simulink model "DroneFlight"  (Simulink 8.0)
settings: Solver=ode4  SolverType=Fixed-step  StopTime=9  FixedStep=drone.step_s
InitFcn:
  | setup_flight;
undefined symbols (not defined in the file): drone
settings Model: ReturnWorkspaceOutputs=on

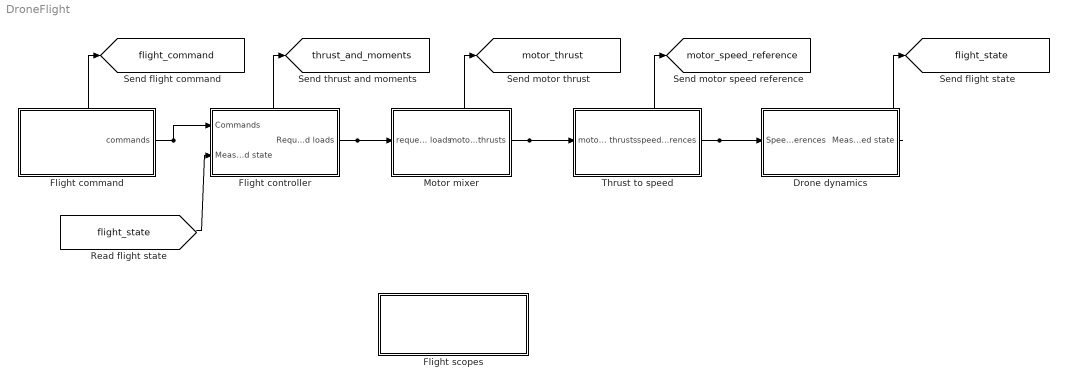
== system DroneFlight ==
  Flight command : Subsystem
  Flight controller : Subsystem
  Motor mixer : Subsystem
  Thrust to speed : Subsystem
  Drone dynamics : Subsystem
  Flight scopes : Subsystem
  tag scope: flight_command=global, flight_state=global, motor_speed_reference=global, motor_thrust=global, thrust_and_moments=global
  wires:
  Flight command/1(commands) -> Flight controller/1(Commands), [flight_command]
  Flight controller/1(Requested loads) -> Motor mixer/1(requested loads), [thrust_and_moments]
  Motor mixer/1(motor thrusts) -> Thrust to speed/1(motor thrusts), [motor_thrust]
  Thrust to speed/1(speed references) -> Drone dynamics/1(Speed references), [motor_speed_reference]
  Drone dynamics/1(Measured state) -> [flight_state]
  [flight_state] -> Flight controller/2(Measured state)

== system DroneFlight/Flight command ==
  Forward speed command : FromWorkspace  VariableName=forward_command  Interpolate=off  OutputAfterFinalValue=Holding final value  SampleTime=drone.step_s
  Right climb height and yaw : FromWorkspace  VariableName=mission_commands  Interpolate=off  OutputAfterFinalValue=Holding final value  SampleTime=drone.step_s
  Collect commands : Mux  Inputs=2
  commands : Outport  Port=1
  wires:
  Forward speed command/1 -> Collect commands/1  "Forward speed (m per s)"
  Right climb height and yaw/1 -> Collect commands/2
  Collect commands/1 -> commands/1

== system DroneFlight/Flight controller ==
  Commands : Inport  Port=1
  Measured state : Inport  Port=2
  Movement references : Demux  Outputs=[2 1 1 1]
  Feedback channels : Demux  Outputs=[2 1 2 1 2 1 3 4]
  Feedback channels unused 1 : Terminator
  Feedback channels unused 8 : Terminator
  Horizontal velocity : Subsystem
  Height and climb : Subsystem
  Attitude and body rates : Subsystem
  Collective roll pitch yaw : Mux  Inputs=2
  Requested loads : Outport  Port=1
  wires:
  Commands/1 -> Movement references/1
  Measured state/1 -> Feedback channels/1
  Feedback channels/1 -> Feedback channels unused 1/1
  Feedback channels/8 -> Feedback channels unused 8/1
  Movement references/1 -> Horizontal velocity/1(Forward and right demand)
  Feedback channels/3 -> Horizontal velocity/2(North and east velocity)
  Feedback channels/6 -> Horizontal velocity/3(Heading)
  Movement references/2 -> Height and climb/1(Climb demand)
  Movement references/3 -> Height and climb/2(Height demand)
  Feedback channels/2 -> Height and climb/3(Down position)
  Feedback channels/4 -> Height and climb/4(Down velocity)
  Feedback channels/5 -> Height and climb/5(Roll and pitch), Attitude and body rates/2(Measured roll and pitch)
  Horizontal velocity/1(Roll and pitch demand) -> Attitude and body rates/1(Demanded roll and pitch)
  Movement references/4 -> Attitude and body rates/3(Demanded yaw rate)
  Feedback channels/7 -> Attitude and body rates/4(Body rates)
  Height and climb/1(Collective thrust) -> Collective roll pitch yaw/1
  Attitude and body rates/1(Body moments) -> Collective roll pitch yaw/2
  Collective roll pitch yaw/1 -> Requested loads/1

== system DroneFlight/Motor mixer ==
  requested loads : Inport  Port=1
  Mix thrust and moments : Gain  Gain=drone.allocation  Multiplication=Matrix(K*u)
  Rotor thrust limits : Subsystem
  motor thrusts : Outport  Port=1
  wires:
  requested loads/1 -> Mix thrust and moments/1
  Mix thrust and moments/1 -> Rotor thrust limits/1(Raw rotor thrusts)
  Rotor thrust limits/1(Feasible thrusts) -> motor thrusts/1

== system DroneFlight/Thrust to speed ==
  motor thrusts : Inport  Port=1
  Inverse thrust coefficient : Gain  Gain=1/drone.kT
  Square root : Sqrt
  speed references : Outport  Port=1
  wires:
  motor thrusts/1 -> Inverse thrust coefficient/1
  Inverse thrust coefficient/1 -> Square root/1
  Square root/1 -> speed references/1

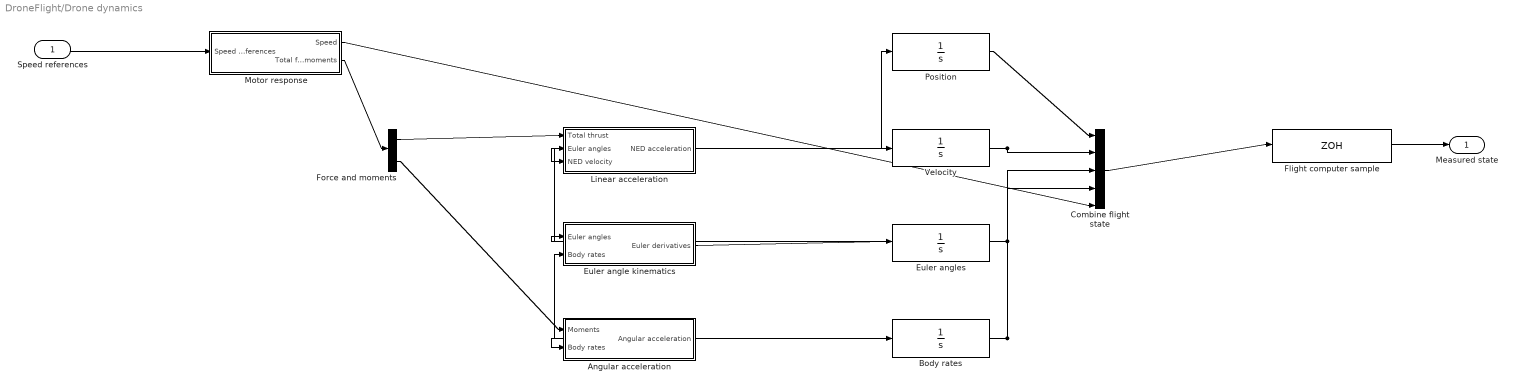
== system DroneFlight/Drone dynamics ==
  Speed references : Inport  Port=1
  Motor response : Subsystem
  Force and moments : Demux  Outputs=[1 3]
  Position : Integrator  InitialCondition=drone.x0(1:3)
  Velocity : Integrator  InitialCondition=drone.x0(4:6)
  Euler angles : Integrator  InitialCondition=drone.x0(7:9)
  Body rates : Integrator  InitialCondition=drone.x0(10:12)
  Linear acceleration : Subsystem
  Euler angle kinematics : Subsystem
  Angular acceleration : Subsystem
  Combine flight state : Mux  Inputs=5
  Flight computer sample : ZeroOrderHold  SampleTime=drone.step_s
  Measured state : Outport  Port=1
  wires:
  Speed references/1 -> Motor response/1(Speed references)
  Motor response/2(Total force and moments) -> Force and moments/1
  Force and moments/1 -> Linear acceleration/1(Total thrust)
  Euler angles/1 -> Linear acceleration/2(Euler angles), Euler angle kinematics/1(Euler angles), Combine flight state/3
  Velocity/1 -> Linear acceleration/3(NED velocity), Position/1, Combine flight state/2
  Body rates/1 -> Euler angle kinematics/2(Body rates), Angular acceleration/2(Body rates), Combine flight state/4
  Force and moments/2 -> Angular acceleration/1(Moments)
  Linear acceleration/1(NED acceleration) -> Velocity/1
  Euler angle kinematics/1(Euler derivatives) -> Euler angles/1
  Angular acceleration/1(Angular acceleration) -> Body rates/1
  Position/1 -> Combine flight state/1
  Motor response/1(Speed) -> Combine flight state/5
  Combine flight state/1 -> Flight computer sample/1
  Flight computer sample/1 -> Measured state/1

== system DroneFlight/Flight scopes ==
  Flight response : Subsystem
  Mixer inputs : Subsystem
  Motor outputs : Subsystem
  Flight measurements : Subsystem
  wires:
  [flight_command] -> Flight response/1(Reference)
  [flight_state] -> Flight measurements/1(State)
  [thrust_and_moments] -> Mixer inputs/1(Controller request)
  [motor_thrust] -> Motor outputs/1(Thrust references)
  [motor_speed_reference] -> Motor outputs/2(Speed references)
  Flight measurements/1(Measurements) -> Flight response/2(Instruments), Motor outputs/3(Instruments)

== system DroneFlight/Flight controller/Horizontal velocity ==
  Forward and right demand : Inport  Port=1
  North and east velocity : Inport  Port=2
  Heading : Inport  Port=3
  Rotate velocity into body : Subsystem
  Velocity error : Sum  Inputs=+-
  Velocity gain : Gain  Gain=drone.velocity_gain_per_s
  Drag feedforward : Gain  Gain=drone.linear_drag_N_per_m_s/drone.mass_kg
  Requested acceleration : Sum  Inputs=++
  Bound horizontal acceleration : Subsystem
  Convert acceleration to tilt : Subsystem
  Roll and pitch demand : Outport  Port=1
  wires:
  North and east velocity/1 -> Rotate velocity into body/1(Planar components)
  Heading/1 -> Rotate velocity into body/2(Yaw)
  Forward and right demand/1 -> Velocity error/1, Drag feedforward/1
  Rotate velocity into body/1(Rotated vector) -> Velocity error/2
  Velocity error/1 -> Velocity gain/1
  Velocity gain/1 -> Requested acceleration/1
  Drag feedforward/1 -> Requested acceleration/2
  Requested acceleration/1 -> Bound horizontal acceleration/1(Acceleration)
  Bound horizontal acceleration/1(Bounded acceleration) -> Convert acceleration to tilt/1(Forward and right acceleration)
  Convert acceleration to tilt/1(Roll and pitch) -> Roll and pitch demand/1

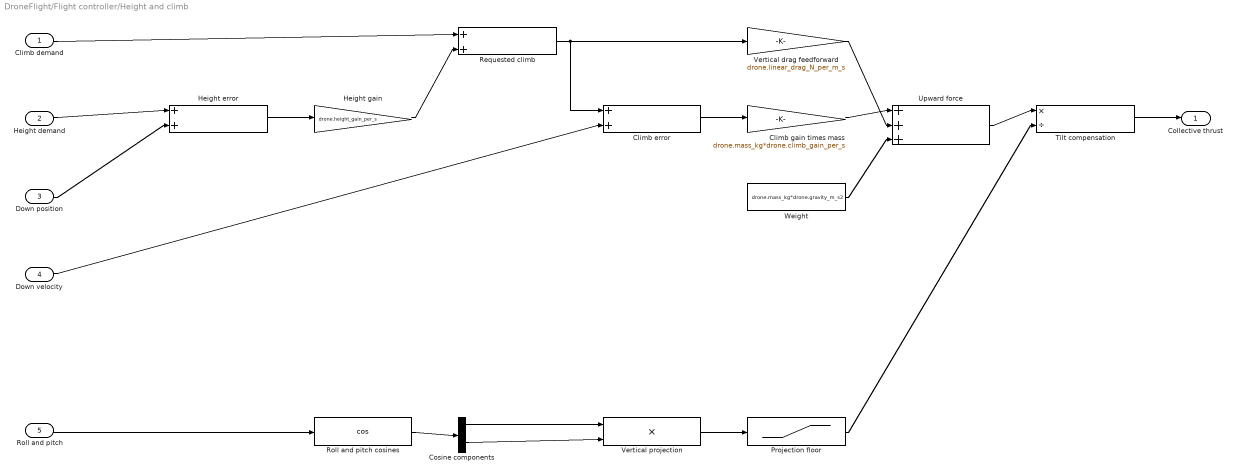
== system DroneFlight/Flight controller/Height and climb ==
  Climb demand : Inport  Port=1
  Height demand : Inport  Port=2
  Down position : Inport  Port=3
  Down velocity : Inport  Port=4
  Roll and pitch : Inport  Port=5
  Height error : Sum  Inputs=++
  Height gain : Gain  Gain=drone.height_gain_per_s
  Requested climb : Sum  Inputs=++
  Climb error : Sum  Inputs=++
  Climb gain times mass : Gain  Gain=drone.mass_kg*drone.climb_gain_per_s
  Vertical drag feedforward : Gain  Gain=drone.linear_drag_N_per_m_s
  Weight : Constant  Value=drone.mass_kg*drone.gravity_m_s2
  Upward force : Sum  Inputs=+++
  Roll and pitch cosines : Trigonometry  Operator=cos
  Cosine components : Demux  Outputs=[1 1]
  Vertical projection : Product  Inputs=**
  Projection floor : Saturate  LowerLimit=0.5  UpperLimit=1
  Tilt compensation : Product  Inputs=*/
  Collective thrust : Outport  Port=1
  wires:
  Height demand/1 -> Height error/1
  Down position/1 -> Height error/2
  Height error/1 -> Height gain/1
  Climb demand/1 -> Requested climb/1
  Height gain/1 -> Requested climb/2
  Requested climb/1 -> Climb error/1, Vertical drag feedforward/1
  Down velocity/1 -> Climb error/2
  Climb error/1 -> Climb gain times mass/1
  Climb gain times mass/1 -> Upward force/1
  Vertical drag feedforward/1 -> Upward force/2
  Weight/1 -> Upward force/3
  Roll and pitch/1 -> Roll and pitch cosines/1
  Roll and pitch cosines/1 -> Cosine components/1
  Cosine components/1 -> Vertical projection/1
  Cosine components/2 -> Vertical projection/2
  Vertical projection/1 -> Projection floor/1
  Upward force/1 -> Tilt compensation/1
  Projection floor/1 -> Tilt compensation/2
  Tilt compensation/1 -> Collective thrust/1

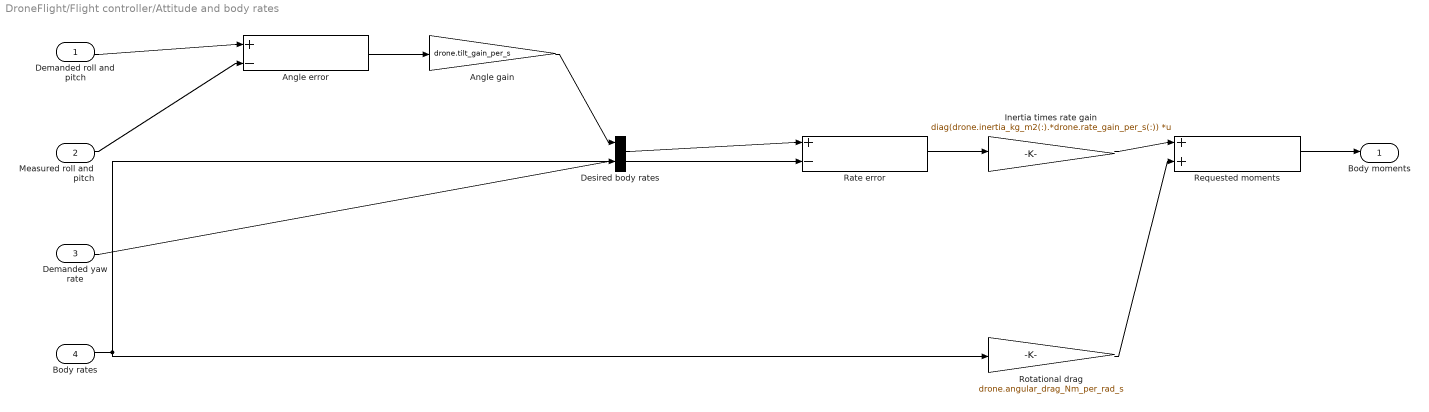
== system DroneFlight/Flight controller/Attitude and body rates ==
  Demanded roll and pitch : Inport  Port=1
  Measured roll and pitch : Inport  Port=2
  Demanded yaw rate : Inport  Port=3
  Body rates : Inport  Port=4
  Angle error : Sum  Inputs=+-
  Angle gain : Gain  Gain=drone.tilt_gain_per_s
  Desired body rates : Mux  Inputs=2
  Rate error : Sum  Inputs=+-
  Inertia times rate gain : Gain  Gain=diag(drone.inertia_kg_m2(:).*drone.rate_gain_per_s(:))  Multiplication=Matrix(K*u)
  Rotational drag : Gain  Gain=drone.angular_drag_Nm_per_rad_s
  Requested moments : Sum  Inputs=++
  Body moments : Outport  Port=1
  wires:
  Demanded roll and pitch/1 -> Angle error/1
  Measured roll and pitch/1 -> Angle error/2
  Angle error/1 -> Angle gain/1
  Angle gain/1 -> Desired body rates/1
  Demanded yaw rate/1 -> Desired body rates/2
  Desired body rates/1 -> Rate error/1
  Body rates/1 -> Rate error/2, Rotational drag/1
  Rate error/1 -> Inertia times rate gain/1
  Inertia times rate gain/1 -> Requested moments/1
  Rotational drag/1 -> Requested moments/2
  Requested moments/1 -> Body moments/1

== system DroneFlight/Motor mixer/Rotor thrust limits ==
  Raw rotor thrusts : Inport  Port=1
  Mean rotor thrust : Gain  Gain=ones(1,4)/4  Multiplication=Matrix(K*u)
  Available collective : Saturate  LowerLimit=0  UpperLimit=drone.max_thrust
  Differential thrusts : Sum  Inputs=+-
  Scale to motor limits : Subsystem
  Scale differences : Product  Inputs=**
  Restore collective : Sum  Inputs=++
  Thrust bounds : Saturate  LowerLimit=0  UpperLimit=drone.max_thrust
  Feasible thrusts : Outport  Port=1
  wires:
  Raw rotor thrusts/1 -> Mean rotor thrust/1, Differential thrusts/1
  Mean rotor thrust/1 -> Available collective/1, Differential thrusts/2
  Differential thrusts/1 -> Scale to motor limits/1(Differential thrusts), Scale differences/1
  Available collective/1 -> Scale to motor limits/2(Collective per rotor), Restore collective/1
  Scale to motor limits/1(Scale) -> Scale differences/2
  Scale differences/1 -> Restore collective/2
  Restore collective/1 -> Thrust bounds/1
  Thrust bounds/1 -> Feasible thrusts/1

== system DroneFlight/Drone dynamics/Motor response ==
  Speed references : Inport  Port=1
  Rotor speed : Integrator  InitialCondition=drone.x0(13:16)
  Speed error : Sum  Inputs=+-
  Inverse motor time constant : Gain  Gain=1/drone.speed_lag_s
  Speed : Outport  Port=1
  Speed squared : Product  Inputs=**
  Propeller thrust : Gain  Gain=drone.kT
  Thrust to body loads : Gain  Gain=drone.effectiveness  Multiplication=Matrix(K*u)
  Total force and moments : Outport  Port=2
  wires:
  Speed references/1 -> Speed error/1
  Rotor speed/1 -> Speed error/2, Speed/1, Speed squared/1, Speed squared/2
  Speed error/1 -> Inverse motor time constant/1
  Inverse motor time constant/1 -> Rotor speed/1
  Speed squared/1 -> Propeller thrust/1
  Propeller thrust/1 -> Thrust to body loads/1
  Thrust to body loads/1 -> Total force and moments/1

== system DroneFlight/Drone dynamics/Linear acceleration ==
  Total thrust : Inport  Port=1
  Euler angles : Inport  Port=2
  NED velocity : Inport  Port=3
  Body thrust direction : Subsystem
  Thrust along body down : Product  Inputs=**
  Linear drag : Gain  Gain=drone.linear_drag_N_per_m_s
  Thrust and drag : Sum  Inputs=++
  Force to acceleration : Gain  Gain=1/drone.mass_kg
  NED gravity : Constant  Value=[0;0;drone.gravity_m_s2]
  Gravity minus thrust and drag : Sum  Inputs=+-
  NED acceleration : Outport  Port=1
  wires:
  Euler angles/1 -> Body thrust direction/1(Euler angles)
  Total thrust/1 -> Thrust along body down/1
  Body thrust direction/1(Body down axis in NED) -> Thrust along body down/2
  NED velocity/1 -> Linear drag/1
  Thrust along body down/1 -> Thrust and drag/1
  Linear drag/1 -> Thrust and drag/2
  Thrust and drag/1 -> Force to acceleration/1
  NED gravity/1 -> Gravity minus thrust and drag/1
  Force to acceleration/1 -> Gravity minus thrust and drag/2
  Gravity minus thrust and drag/1 -> NED acceleration/1

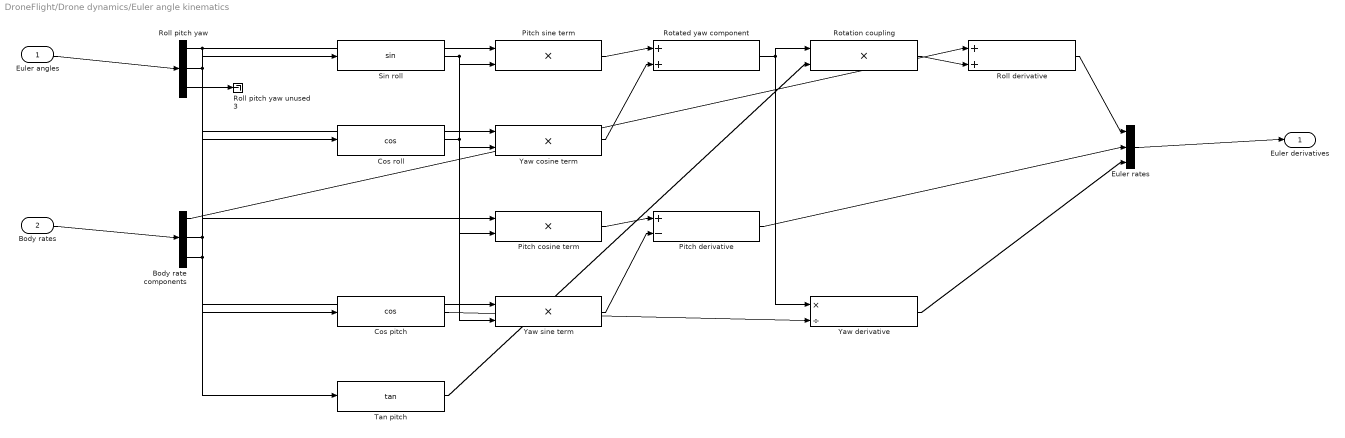
== system DroneFlight/Drone dynamics/Euler angle kinematics ==
  Euler angles : Inport  Port=1
  Body rates : Inport  Port=2
  Roll pitch yaw : Demux  Outputs=[1 1 1]
  Roll pitch yaw unused 3 : Terminator
  Body rate components : Demux  Outputs=[1 1 1]
  Sin roll : Trigonometry  Operator=sin
  Cos roll : Trigonometry  Operator=cos
  Cos pitch : Trigonometry  Operator=cos
  Tan pitch : Trigonometry  Operator=tan
  Pitch sine term : Product  Inputs=**
  Yaw cosine term : Product  Inputs=**
  Pitch cosine term : Product  Inputs=**
  Yaw sine term : Product  Inputs=**
  Rotated yaw component : Sum  Inputs=++
  Pitch derivative : Sum  Inputs=+-
  Rotation coupling : Product  Inputs=**
  Yaw derivative : Product  Inputs=*/
  Roll derivative : Sum  Inputs=++
  Euler rates : Mux  Inputs=3
  Euler derivatives : Outport  Port=1
  wires:
  Euler angles/1 -> Roll pitch yaw/1
  Roll pitch yaw/3 -> Roll pitch yaw unused 3/1
  Body rates/1 -> Body rate components/1
  Roll pitch yaw/1 -> Sin roll/1, Cos roll/1
  Roll pitch yaw/2 -> Cos pitch/1, Tan pitch/1
  Body rate components/2 -> Pitch sine term/1, Pitch cosine term/1
  Sin roll/1 -> Pitch sine term/2, Yaw sine term/2
  Body rate components/3 -> Yaw cosine term/1, Yaw sine term/1
  Cos roll/1 -> Yaw cosine term/2, Pitch cosine term/2
  Pitch sine term/1 -> Rotated yaw component/1
  Yaw cosine term/1 -> Rotated yaw component/2
  Pitch cosine term/1 -> Pitch derivative/1
  Yaw sine term/1 -> Pitch derivative/2
  Rotated yaw component/1 -> Rotation coupling/1, Yaw derivative/1
  Tan pitch/1 -> Rotation coupling/2
  Cos pitch/1 -> Yaw derivative/2
  Body rate components/1 -> Roll derivative/1
  Rotation coupling/1 -> Roll derivative/2
  Roll derivative/1 -> Euler rates/1
  Pitch derivative/1 -> Euler rates/2
  Yaw derivative/1 -> Euler rates/3
  Euler rates/1 -> Euler derivatives/1

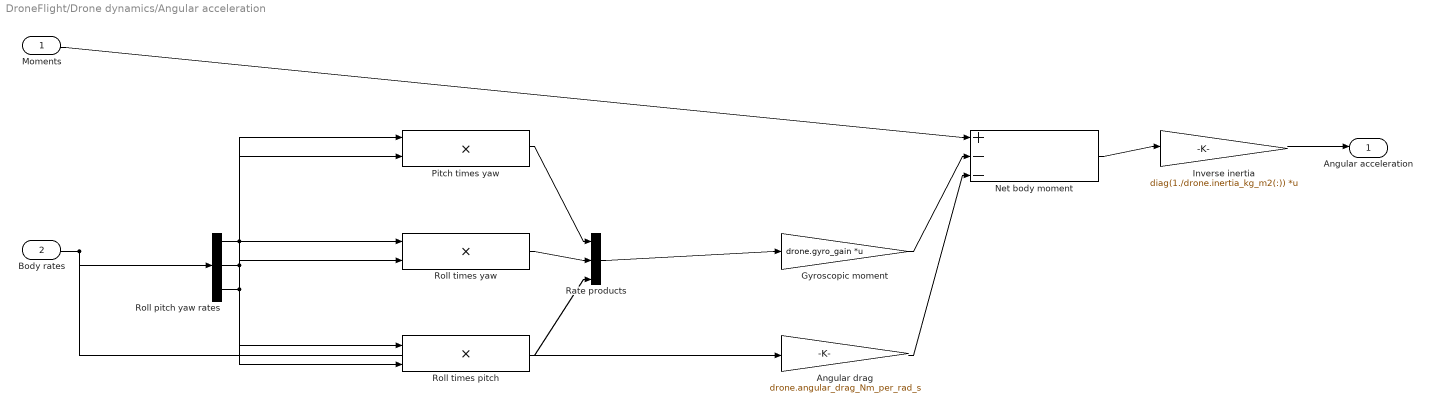
== system DroneFlight/Drone dynamics/Angular acceleration ==
  Moments : Inport  Port=1
  Body rates : Inport  Port=2
  Roll pitch yaw rates : Demux  Outputs=[1 1 1]
  Pitch times yaw : Product  Inputs=**
  Roll times yaw : Product  Inputs=**
  Roll times pitch : Product  Inputs=**
  Rate products : Mux  Inputs=3
  Gyroscopic moment : Gain  Gain=drone.gyro_gain  Multiplication=Matrix(K*u)
  Angular drag : Gain  Gain=drone.angular_drag_Nm_per_rad_s
  Net body moment : Sum  Inputs=+--
  Inverse inertia : Gain  Gain=diag(1./drone.inertia_kg_m2(:))  Multiplication=Matrix(K*u)
  Angular acceleration : Outport  Port=1
  wires:
  Body rates/1 -> Roll pitch yaw rates/1, Angular drag/1
  Roll pitch yaw rates/2 -> Pitch times yaw/1, Roll times pitch/2
  Roll pitch yaw rates/3 -> Pitch times yaw/2, Roll times yaw/2
  Roll pitch yaw rates/1 -> Roll times yaw/1, Roll times pitch/1
  Pitch times yaw/1 -> Rate products/1
  Roll times yaw/1 -> Rate products/2
  Roll times pitch/1 -> Rate products/3
  Rate products/1 -> Gyroscopic moment/1
  Moments/1 -> Net body moment/1
  Gyroscopic moment/1 -> Net body moment/2
  Angular drag/1 -> Net body moment/3
  Net body moment/1 -> Inverse inertia/1
  Inverse inertia/1 -> Angular acceleration/1

== system DroneFlight/Flight scopes/Flight response ==
  Reference : Inport  Port=1
  Instruments : Inport  Port=2
  Reference channels : Demux  Outputs=[1 2 1 1]
  Reference channels unused 2 : Terminator
  Reference channels unused 4 : Terminator
  Measured channels : Demux  Outputs=[1 1 2 3 8]
  Measured channels unused 5 : Terminator
  Forward speed - m per s : Scope  NumInputPorts=2
      settings: OpenAtSimulationStart=off
  Height - m : Scope  NumInputPorts=2
      settings: OpenAtSimulationStart=off
  North and east - m : Scope
      settings: OpenAtSimulationStart=off
  Roll pitch yaw - deg : Scope
      settings: OpenAtSimulationStart=off
  wires:
  Reference/1 -> Reference channels/1
  Reference channels/2 -> Reference channels unused 2/1
  Reference channels/4 -> Reference channels unused 4/1
  Instruments/1 -> Measured channels/1
  Measured channels/5 -> Measured channels unused 5/1
  Reference channels/1 -> Forward speed - m per s/1  "Command"
  Measured channels/1 -> Forward speed - m per s/2  "Actual"
  Reference channels/3 -> Height - m/1  "Target height"
  Measured channels/2 -> Height - m/2  "Measured height"
  Measured channels/3 -> North and east - m/1
  Measured channels/4 -> Roll pitch yaw - deg/1

== system DroneFlight/Flight scopes/Mixer inputs ==
  Controller request : Inport  Port=1
  Force and moments : Demux  Outputs=[1 3]
  Collective thrust - N : Scope
      settings: OpenAtSimulationStart=off
  Roll pitch yaw moments - Nm : Scope
      settings: OpenAtSimulationStart=off
  wires:
  Controller request/1 -> Force and moments/1
  Force and moments/1 -> Collective thrust - N/1
  Force and moments/2 -> Roll pitch yaw moments - Nm/1

== system DroneFlight/Flight scopes/Motor outputs ==
  Thrust references : Inport  Port=1
  Speed references : Inport  Port=2
  Instruments : Inport  Port=3
  Four thrust references - N channels : Demux  Outputs=[1 1 1 1]
  Four thrust references - N : Scope  NumInputPorts=4
      settings: OpenAtSimulationStart=off
  Radians per second to rpm : Gain  Gain=30/pi
  Four speed references - rpm channels : Demux  Outputs=[1 1 1 1]
  Four speed references - rpm : Scope  NumInputPorts=4
      settings: OpenAtSimulationStart=off
  Motor measurements : Demux  Outputs=[7 4 4]
  Motor measurements unused 1 : Terminator
  Actual rotor speeds - rpm : Scope
      settings: OpenAtSimulationStart=off
  Propeller loads - Nm : Scope
      settings: OpenAtSimulationStart=off
  wires:
  Thrust references/1 -> Four thrust references - N channels/1
  Four thrust references - N channels/1 -> Four thrust references - N/1  "M1 front right N"
  Four thrust references - N channels/2 -> Four thrust references - N/2  "M2 back left N"
  Four thrust references - N channels/3 -> Four thrust references - N/3  "M3 front left N"
  Four thrust references - N channels/4 -> Four thrust references - N/4  "M4 back right N"
  Speed references/1 -> Radians per second to rpm/1
  Radians per second to rpm/1 -> Four speed references - rpm channels/1
  Four speed references - rpm channels/1 -> Four speed references - rpm/1  "M1 front right rpm"
  Four speed references - rpm channels/2 -> Four speed references - rpm/2  "M2 back left rpm"
  Four speed references - rpm channels/3 -> Four speed references - rpm/3  "M3 front left rpm"
  Four speed references - rpm channels/4 -> Four speed references - rpm/4  "M4 back right rpm"
  Instruments/1 -> Motor measurements/1
  Motor measurements/1 -> Motor measurements unused 1/1
  Motor measurements/2 -> Actual rotor speeds - rpm/1
  Motor measurements/3 -> Propeller loads - Nm/1

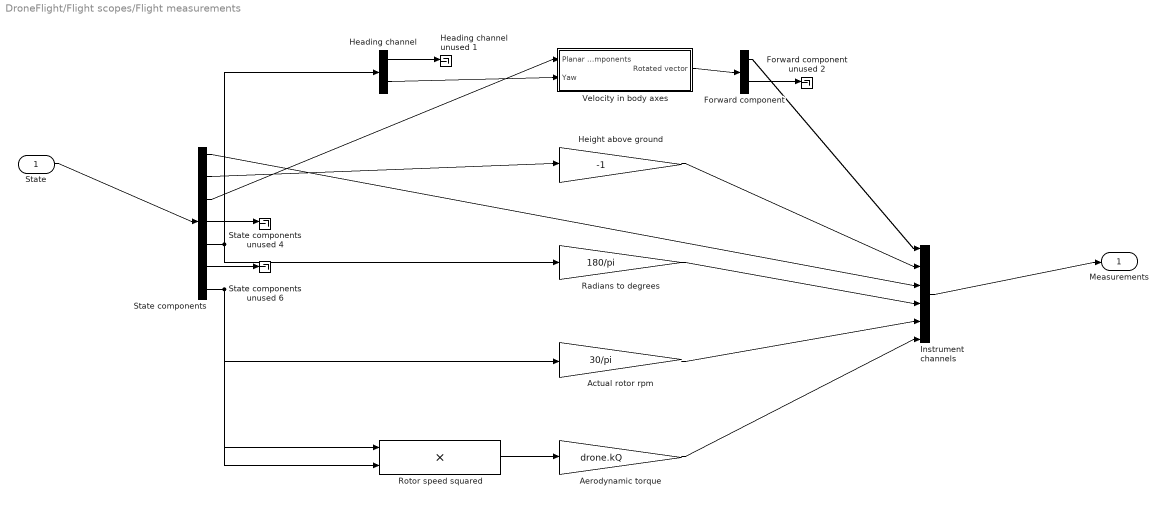
== system DroneFlight/Flight scopes/Flight measurements ==
  State : Inport  Port=1
  State components : Demux  Outputs=[2 1 2 1 3 3 4]
  State components unused 4 : Terminator
  State components unused 6 : Terminator
  Heading channel : Demux  Outputs=[2 1]
  Heading channel unused 1 : Terminator
  Velocity in body axes : Subsystem
  Forward component : Demux  Outputs=[1 1]
  Forward component unused 2 : Terminator
  Height above ground : Gain  Gain=-1
  Radians to degrees : Gain  Gain=180/pi
  Actual rotor rpm : Gain  Gain=30/pi
  Rotor speed squared : Product  Inputs=**
  Aerodynamic torque : Gain  Gain=drone.kQ
  Instrument channels : Mux  Inputs=6
  Measurements : Outport  Port=1
  wires:
  State/1 -> State components/1
  State components/4 -> State components unused 4/1
  State components/6 -> State components unused 6/1
  State components/5 -> Heading channel/1, Radians to degrees/1
  Heading channel/1 -> Heading channel unused 1/1
  State components/3 -> Velocity in body axes/1(Planar components)
  Heading channel/2 -> Velocity in body axes/2(Yaw)
  Velocity in body axes/1(Rotated vector) -> Forward component/1
  Forward component/2 -> Forward component unused 2/1
  State components/2 -> Height above ground/1
  State components/7 -> Actual rotor rpm/1, Rotor speed squared/1, Rotor speed squared/2
  Rotor speed squared/1 -> Aerodynamic torque/1
  Forward component/1 -> Instrument channels/1
  Height above ground/1 -> Instrument channels/2
  State components/1 -> Instrument channels/3
  Radians to degrees/1 -> Instrument channels/4
  Actual rotor rpm/1 -> Instrument channels/5
  Aerodynamic torque/1 -> Instrument channels/6
  Instrument channels/1 -> Measurements/1

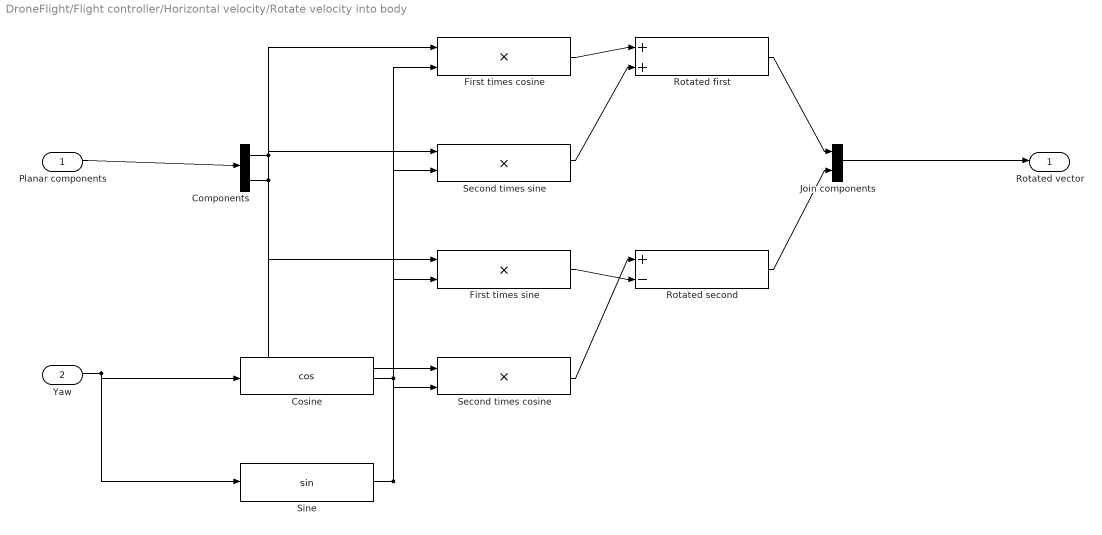
== system DroneFlight/Flight controller/Horizontal velocity/Rotate velocity into body ==
  Planar components : Inport  Port=1
  Components : Demux  Outputs=[1 1]
  Yaw : Inport  Port=2
  Cosine : Trigonometry  Operator=cos
  Sine : Trigonometry  Operator=sin
  First times cosine : Product  Inputs=**
  Second times sine : Product  Inputs=**
  First times sine : Product  Inputs=**
  Second times cosine : Product  Inputs=**
  Rotated first : Sum  Inputs=++
  Rotated second : Sum  Inputs=+-
  Join components : Mux  Inputs=2
  Rotated vector : Outport  Port=1
  wires:
  Planar components/1 -> Components/1
  Yaw/1 -> Cosine/1, Sine/1
  Components/1 -> First times cosine/1, First times sine/1
  Cosine/1 -> First times cosine/2, Second times cosine/2
  Components/2 -> Second times sine/1, Second times cosine/1
  Sine/1 -> Second times sine/2, First times sine/2
  First times cosine/1 -> Rotated first/1
  Second times sine/1 -> Rotated first/2
  Second times cosine/1 -> Rotated second/1
  First times sine/1 -> Rotated second/2
  Rotated first/1 -> Join components/1
  Rotated second/1 -> Join components/2
  Join components/1 -> Rotated vector/1

== system DroneFlight/Flight controller/Horizontal velocity/Bound horizontal acceleration ==
  Acceleration : Inport  Port=1
  Squared magnitude : DotProduct
  Magnitude : Sqrt
  Relative to limit : Gain  Gain=1/drone.max_accel_m_s2
  Minimum divisor of one : Saturate  LowerLimit=1  UpperLimit=inf
  Scale vector : Product  Inputs=*/
  Bounded acceleration : Outport  Port=1
  wires:
  Acceleration/1 -> Squared magnitude/1, Squared magnitude/2, Scale vector/1
  Squared magnitude/1 -> Magnitude/1
  Magnitude/1 -> Relative to limit/1
  Relative to limit/1 -> Minimum divisor of one/1
  Minimum divisor of one/1 -> Scale vector/2
  Scale vector/1 -> Bounded acceleration/1

== system DroneFlight/Flight controller/Horizontal velocity/Convert acceleration to tilt ==
  Forward and right acceleration : Inport  Port=1
  Divide by gravity : Gain  Gain=1/drone.gravity_m_s2
  Tilt angles : Trigonometry  Operator=atan
  Right to roll and forward to pitch : Gain  Gain=[0 1;-1 0]  Multiplication=Matrix(K*u)
  Roll and pitch : Outport  Port=1
  wires:
  Forward and right acceleration/1 -> Divide by gravity/1
  Divide by gravity/1 -> Tilt angles/1
  Tilt angles/1 -> Right to roll and forward to pitch/1
  Right to roll and forward to pitch/1 -> Roll and pitch/1

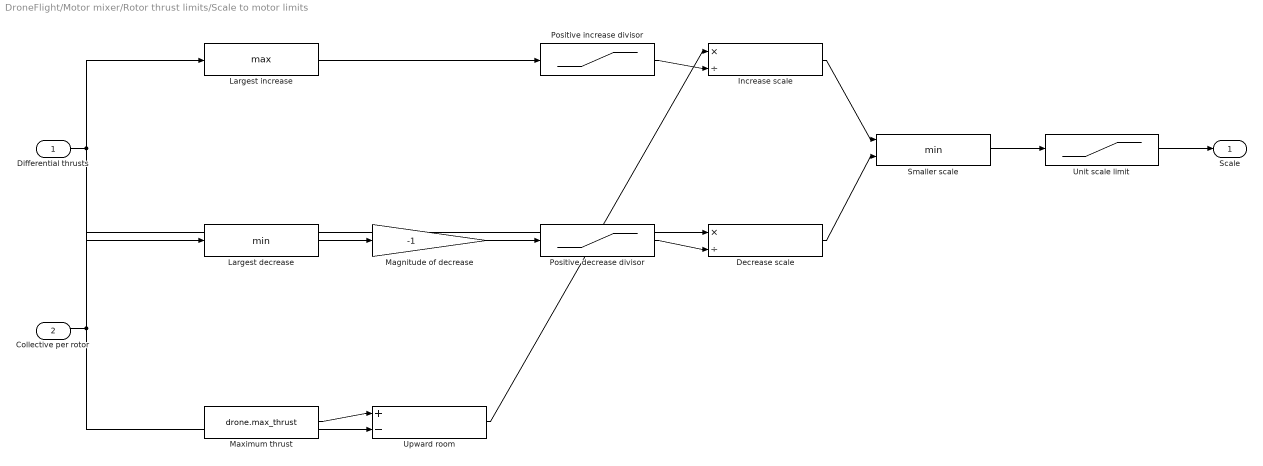
== system DroneFlight/Motor mixer/Rotor thrust limits/Scale to motor limits ==
  Differential thrusts : Inport  Port=1
  Collective per rotor : Inport  Port=2
  Largest increase : MinMax  Function=max  Inputs=1
  Largest decrease : MinMax  Function=min  Inputs=1
  Magnitude of decrease : Gain  Gain=-1
  Maximum thrust : Constant  Value=drone.max_thrust
  Upward room : Sum  Inputs=+-
  Positive increase divisor : Saturate  LowerLimit=eps  UpperLimit=inf
  Positive decrease divisor : Saturate  LowerLimit=eps  UpperLimit=inf
  Increase scale : Product  Inputs=*/
  Decrease scale : Product  Inputs=*/
  Smaller scale : MinMax  Function=min  Inputs=2
  Unit scale limit : Saturate  LowerLimit=0  UpperLimit=1
  Scale : Outport  Port=1
  wires:
  Differential thrusts/1 -> Largest increase/1, Largest decrease/1
  Largest decrease/1 -> Magnitude of decrease/1
  Maximum thrust/1 -> Upward room/1
  Collective per rotor/1 -> Upward room/2, Decrease scale/1
  Largest increase/1 -> Positive increase divisor/1
  Magnitude of decrease/1 -> Positive decrease divisor/1
  Upward room/1 -> Increase scale/1
  Positive increase divisor/1 -> Increase scale/2
  Positive decrease divisor/1 -> Decrease scale/2
  Increase scale/1 -> Smaller scale/1
  Decrease scale/1 -> Smaller scale/2
  Smaller scale/1 -> Unit scale limit/1
  Unit scale limit/1 -> Scale/1

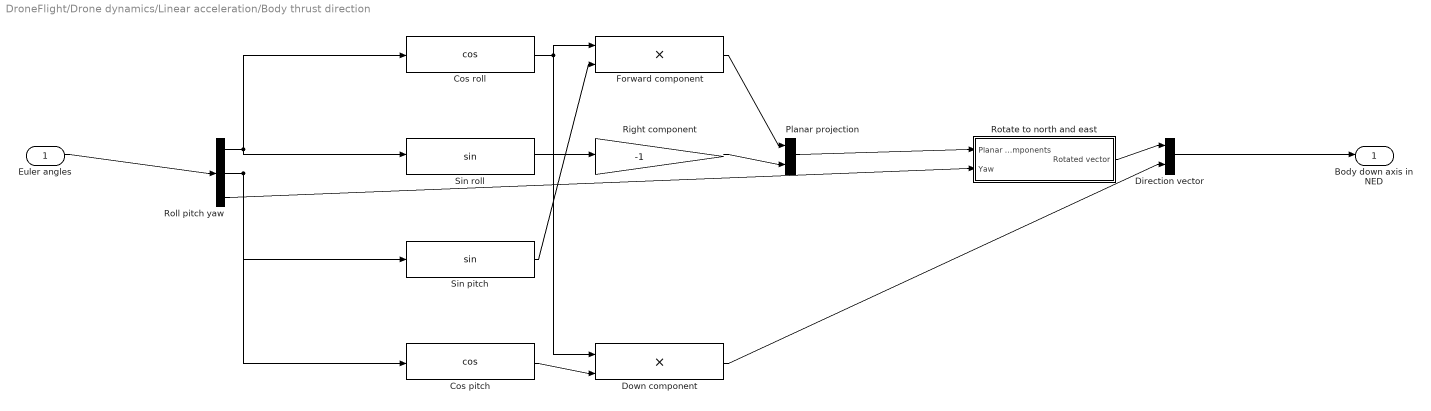
== system DroneFlight/Drone dynamics/Linear acceleration/Body thrust direction ==
  Euler angles : Inport  Port=1
  Roll pitch yaw : Demux  Outputs=[1 1 1]
  Cos roll : Trigonometry  Operator=cos
  Sin roll : Trigonometry  Operator=sin
  Sin pitch : Trigonometry  Operator=sin
  Cos pitch : Trigonometry  Operator=cos
  Forward component : Product  Inputs=**
  Right component : Gain  Gain=-1
  Down component : Product  Inputs=**
  Planar projection : Mux  Inputs=2
  Rotate to north and east : Subsystem
  Direction vector : Mux  Inputs=2
  Body down axis in NED : Outport  Port=1
  wires:
  Euler angles/1 -> Roll pitch yaw/1
  Roll pitch yaw/1 -> Cos roll/1, Sin roll/1
  Roll pitch yaw/2 -> Sin pitch/1, Cos pitch/1
  Cos roll/1 -> Forward component/1, Down component/1
  Sin pitch/1 -> Forward component/2
  Sin roll/1 -> Right component/1
  Cos pitch/1 -> Down component/2
  Forward component/1 -> Planar projection/1
  Right component/1 -> Planar projection/2
  Planar projection/1 -> Rotate to north and east/1(Planar components)
  Roll pitch yaw/3 -> Rotate to north and east/2(Yaw)
  Rotate to north and east/1(Rotated vector) -> Direction vector/1
  Down component/1 -> Direction vector/2
  Direction vector/1 -> Body down axis in NED/1

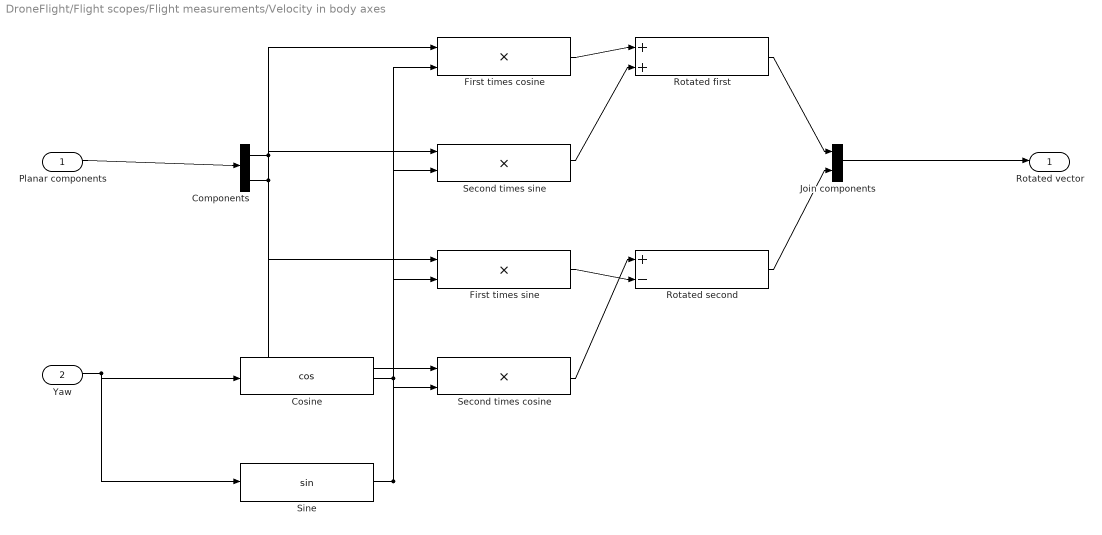
== system DroneFlight/Flight scopes/Flight measurements/Velocity in body axes ==
  Planar components : Inport  Port=1
  Components : Demux  Outputs=[1 1]
  Yaw : Inport  Port=2
  Cosine : Trigonometry  Operator=cos
  Sine : Trigonometry  Operator=sin
  First times cosine : Product  Inputs=**
  Second times sine : Product  Inputs=**
  First times sine : Product  Inputs=**
  Second times cosine : Product  Inputs=**
  Rotated first : Sum  Inputs=++
  Rotated second : Sum  Inputs=+-
  Join components : Mux  Inputs=2
  Rotated vector : Outport  Port=1
  wires:
  Planar components/1 -> Components/1
  Yaw/1 -> Cosine/1, Sine/1
  Components/1 -> First times cosine/1, First times sine/1
  Cosine/1 -> First times cosine/2, Second times cosine/2
  Components/2 -> Second times sine/1, Second times cosine/1
  Sine/1 -> Second times sine/2, First times sine/2
  First times cosine/1 -> Rotated first/1
  Second times sine/1 -> Rotated first/2
  Second times cosine/1 -> Rotated second/1
  First times sine/1 -> Rotated second/2
  Rotated first/1 -> Join components/1
  Rotated second/1 -> Join components/2
  Join components/1 -> Rotated vector/1

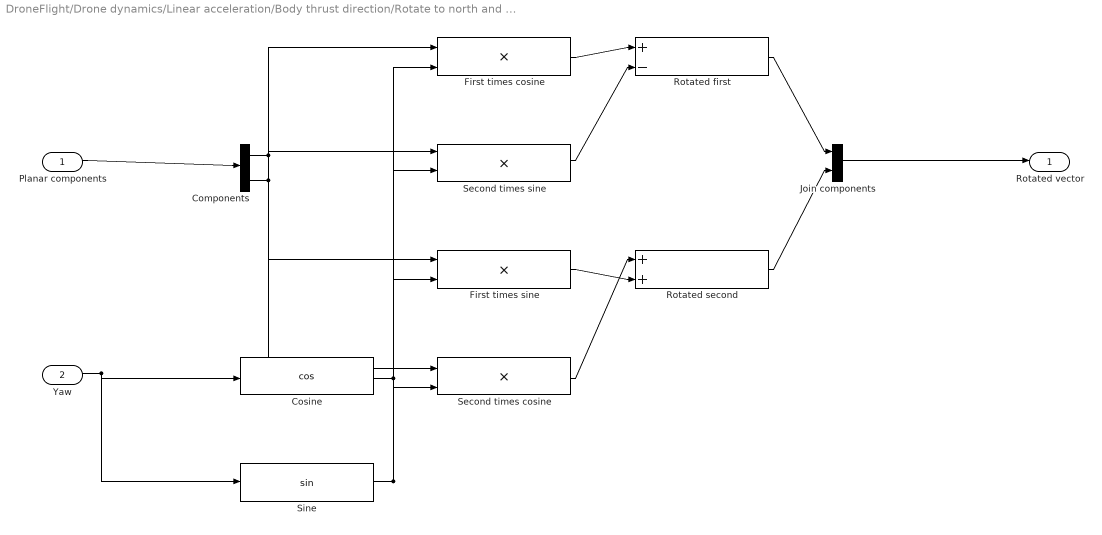
== system DroneFlight/Drone dynamics/Linear acceleration/Body thrust direction/Rotate to north and east ==
  Planar components : Inport  Port=1
  Components : Demux  Outputs=[1 1]
  Yaw : Inport  Port=2
  Cosine : Trigonometry  Operator=cos
  Sine : Trigonometry  Operator=sin
  First times cosine : Product  Inputs=**
  Second times sine : Product  Inputs=**
  First times sine : Product  Inputs=**
  Second times cosine : Product  Inputs=**
  Rotated first : Sum  Inputs=+-
  Rotated second : Sum  Inputs=++
  Join components : Mux  Inputs=2
  Rotated vector : Outport  Port=1
  wires:
  Planar components/1 -> Components/1
  Yaw/1 -> Cosine/1, Sine/1
  Components/1 -> First times cosine/1, First times sine/1
  Cosine/1 -> First times cosine/2, Second times cosine/2
  Components/2 -> Second times sine/1, Second times cosine/1
  Sine/1 -> Second times sine/2, First times sine/2
  First times cosine/1 -> Rotated first/1
  Second times sine/1 -> Rotated first/2
  Second times cosine/1 -> Rotated second/1
  First times sine/1 -> Rotated second/2
  Rotated first/1 -> Join components/1
  Rotated second/1 -> Join components/2
  Join components/1 -> Rotated vector/1
